simulink model "RobustFormationControl_IntegerModel_under_Dis"  (R2023a)
settings: Solver=ode3  StartTime=0.0  StopTime=30  FixedStep=0.0001  RelTol=1e-3
InitFcn:
  | % % Parameters for the fractional order NTFSMC:
  | % Sliding Surface " Sx, Sy, and Sz ":
  | %------------------------
  | % 10
  | % 10
  | cx = 2*[4 4 4];
  | cxx = 1*[0.01 0.01 0.01];
  | 
  | cx1 = cx(1);
  | cy1 = cx(2);
  | cz1 = cx(3);
  | 
  | cx2 = cxx(1);
  | cy2 = cxx(2);
  | cz2 = cxx(3);
  | 
  | alpha1 = [0.6 0.6 0.6];
  | alpha2 = [0.1 0.1 0.1];
  | 
  | gammaX = [3 3 3];
  | gx  = gammaX(1);
  | gy = gammaX(2);
  | gz = gammaX(3);
  | 
  | p = 10;
  | q = 10;
  | 
  | % Sliding Surface " S_Phi , S_Theta, and  S_Psi":
  | %------------------------
  | cP = 2*[4 4 4];
  | cPP = 1*[0.01 0.01 0.01 0.01];
  | 
  | cPhi1 = cP(1);
  | cTheta1 = cP(2);
  | cPsi1 = cP(3);
  | 
  | cPhi2 = cPP(1);
  | cTheta2 = cPP(2);
  | cPsi2 = cPP(3);
  | gammaP = [3 3 3];
  | 
  | %=========================
  | %=========================
  | SigmaX = 1*[0.01 0.01 0.01];
  | SigmaXX =1*[1 1 1];
  | 
  | Sigma1X = SigmaX(1);
  | Sigma1Y = SigmaX(2);
  | Sigma1Z = SigmaX(3);
  | %-----
  | Sigma2X = SigmaXX(1);
  | Sigma2Y = SigmaXX(2);
  | Sigma2Z = SigmaXX(3);
  | 
  | 
  | SigmaP = 1*[0.01 0.01 0.01];
  | SigmaPP =1*[1 1 1];
  | 
  | Sigma1Phi   = SigmaP(1);
  | Sigma1Theta = SigmaP(2);
  | ... (+80 lines)
values from neighbouring files (symbols this model uses):
  a1 = (Iyy - Izz)/Ixx    (= -0.812397034596)    [init_quadrotor_params.m]
  a2 = (Izz - Ixx)/Iyy    (= 0.812397034596)    [init_quadrotor_params.m]
  a3 = (Ixx - Iyy)/Izz    (= 0)    [init_quadrotor_params.m]
  a4 = - Ktx/m    (= -0.00114547325103)    [init_quadrotor_params.m]
  a5 = - Kty/m    (= -0.00114547325103)    [init_quadrotor_params.m]
  a6 = - Ktz/m    (= -0.00130740740741)    [init_quadrotor_params.m]
  b = 2.980e-5    (= 2.98e-05)    [init_quadrotor_params.m]
  b1 = - Jr/Ixx    (= -0.00584534596376)    [init_quadrotor_params.m]
  b2 = Jr/Iyy    (= 0.00584534596376)    [init_quadrotor_params.m]
  b3 = - Kfz/Izz    (= -0.0721963413248)    [init_quadrotor_params.m]
  b4 = 1/m    (= 2.05761316872)    [init_quadrotor_params.m]
  b5 = 1/m    (= 2.05761316872)    [init_quadrotor_params.m]
  b6 = 1/m    (= 2.05761316872)    [init_quadrotor_params.m]
  c1 = - Kfx/Ixx    (= -0.114641680395)    [init_quadrotor_params.m]
  c2 = - Kfy/Iyy    (= -0.114641680395)    [init_quadrotor_params.m]
  c3 = 1/Izz    (= 113.62345188)    [init_quadrotor_params.m]
  d = 1.12e-06    [init_quadrotor_params.m]
  d1 = L/Ixx    (= 46.334431631)    [init_quadrotor_params.m]
  d2 = L/Iyy    (= 46.334431631)    [init_quadrotor_params.m]
  g = 9.81    [init_quadrotor_params.m]
  Ixx = 4.856e-3    (= 0.004856)    [init_quadrotor_params.m]
  Iyy = 4.856e-3    (= 0.004856)    [init_quadrotor_params.m]
  Izz = 8.801e-3    (= 0.008801)    [init_quadrotor_params.m]
  Jr = 2.8385e-5    (= 2.8385e-05)    [init_quadrotor_params.m]
  Kfx = 5.567e-4    (= 0.0005567)    [init_quadrotor_params.m]
  Kfy = 5.567e-4    (= 0.0005567)    [init_quadrotor_params.m]
  Kfz = 6.354e-4    (= 0.0006354)    [init_quadrotor_params.m]
  Ktx = 5.5670e-4    (= 0.0005567)    [init_quadrotor_params.m]
  Kty = 5.5670e-4    (= 0.0005567)    [init_quadrotor_params.m]
  Ktz = 6.3540e-4    (= 0.0006354)    [init_quadrotor_params.m]
  L = 0.225    [init_quadrotor_params.m]
  m = 0.486    [init_quadrotor_params.m]
libraries: fod x120, eeStairGenerator x5
(part 9 of 9)

== system RobustFormationControl_IntegerModel_under_Dis/Integer Leader and four followers/Leader System/Integer Model/Control Module1/Subsystem/Subsystem1 ==
  Ux : Inport
  Uy : Inport  Port=2
  Psi_d : Inport  Port=3
  Phi_d : Inport  Port=4
  Constant : Constant
  Divide : Product  Inputs=*/
  Product : Product
  Product1 : Product
  Product2 : Product
  Subtract : Sum
  Trigonometric Function : Trigonometry  Operator=cos
  Trigonometric Function1 : Trigonometry
  Trigonometric Function2 : Trigonometry  Operator=asin
  Trigonometric Function3 : Trigonometry  Operator=cos
  Theta_d : Outport  VectorParamsAs1DForOutWhenUnconnected=off
  wires:
  Product1/1 -> Subtract/2
  Uy/1 -> Product1/2
  Ux/1 -> Product/1
  Trigonometric Function1/1 -> Product1/1
  Psi_d/1 -> Trigonometric Function1/1, Trigonometric Function/1
  Product/1 -> Subtract/1
  Trigonometric Function/1 -> Product/2
  Trigonometric Function2/1 -> Theta_d/1
  Constant/1 -> Divide/1
  Product2/1 -> Trigonometric Function2/1
  Subtract/1 -> Product2/1
  Divide/1 -> Product2/2
  Trigonometric Function3/1 -> Divide/2
  Phi_d/1 -> Trigonometric Function3/1

== system RobustFormationControl_IntegerModel_under_Dis/Integer Leader and four followers/Leader System/Integer Model/Control Module1/Subsystem1/Subsystem ==
  x1 : Inport
  xd1 : Inport  Port=2
  x2 : Inport  Port=3
  xd2 : Inport  Port=4
  Constant : Constant  Value=p/q
  Constant1 : Constant  Value=gammaP(1)
  Divide : Product  Inputs=**  RndMeth=Zero  SaturateOnIntegerOverflow=on
  Fractional integrator : fod/Fractional integrator  gam=0.01  ww=[0.001; 1000]  n=5  nFod=off
      settings: SourceProductName=FOMCON Toolbox
  Fractional integrator1 : fod/Fractional integrator  gam=0.01  ww=[0.001; 1000]  n=5  nFod=off
      settings: SourceProductName=FOMCON Toolbox
  Gain : Gain  Gain=cPhi1
  Gain1 : Gain  Gain=cPhi2
  Power : Math  Operator=pow
  Power1 : Math  Operator=pow
  Sign : Signum
  Sum1 : Sum  Inputs=+-
  Sum2 : Sum  Inputs=+++
  Sum3 : Sum  Inputs=+-
  S2 : Outport  VectorParamsAs1DForOutWhenUnconnected=off
  wires:
  xd2/1 -> Sum1/2
  Sum2/1 -> S2/1
  xd1/1 -> Sum3/2
  x1/1 -> Sum3/1
  x2/1 -> Sum1/1
  Sum3/1 -> Power1/1, Sign/1, Power/1
  Constant/1 -> Power/2
  Power/1 -> Gain/1
  Gain/1 -> Fractional integrator/1
  Constant1/1 -> Power1/2
  Sign/1 -> Divide/1
  Power1/1 -> Divide/2
  Divide/1 -> Gain1/1
  Gain1/1 -> Fractional integrator1/1
  Sum1/1 -> Sum2/1
  Fractional integrator/1 -> Sum2/2
  Fractional integrator1/1 -> Sum2/3

== system RobustFormationControl_IntegerModel_under_Dis/Integer Leader and four followers/Leader System/Integer Model/Control Module1/Subsystem1/Subsystem1 ==
  x5 : Inport
  xd5 : Inport  Port=2
  x6 : Inport  Port=3
  xd6 : Inport  Port=4
  Constant : Constant  Value=p/q
  Constant1 : Constant  Value=gammaP(3)
  Divide : Product  Inputs=**  RndMeth=Zero  SaturateOnIntegerOverflow=on
  Fractional integrator : fod/Fractional integrator  gam=0.1  ww=[0.001; 1000]  n=5  nFod=off
      settings: SourceProductName=FOMCON Toolbox
  Fractional integrator1 : fod/Fractional integrator  gam=0.1  ww=[0.001; 1000]  n=5  nFod=off
      settings: SourceProductName=FOMCON Toolbox
  Gain : Gain  Gain=cPsi1
  Gain1 : Gain  Gain=cPsi2
  Power : Math  Operator=pow
  Power1 : Math  Operator=pow
  Sign : Signum
  Sum1 : Sum  Inputs=+-
  Sum2 : Sum  Inputs=+++
  Sum3 : Sum  Inputs=+-
  S6 : Outport  VectorParamsAs1DForOutWhenUnconnected=off
  wires:
  xd6/1 -> Sum1/2
  Sum2/1 -> S6/1
  xd5/1 -> Sum3/2
  x5/1 -> Sum3/1
  x6/1 -> Sum1/1
  Sum3/1 -> Power1/1, Sign/1, Power/1
  Constant/1 -> Power/2
  Power/1 -> Gain/1
  Gain/1 -> Fractional integrator/1
  Constant1/1 -> Power1/2
  Sign/1 -> Divide/1
  Power1/1 -> Divide/2
  Divide/1 -> Gain1/1
  Gain1/1 -> Fractional integrator1/1
  Sum1/1 -> Sum2/1
  Fractional integrator/1 -> Sum2/2
  Fractional integrator1/1 -> Sum2/3

== system RobustFormationControl_IntegerModel_under_Dis/Integer Leader and four followers/Leader System/Integer Model/Control Module1/Subsystem1/Subsystem2 ==
  x7 : Inport
  xd7 : Inport  Port=2
  x8 : Inport  Port=3
  xd8 : Inport  Port=4
  Constant : Constant  Value=p/q
  Constant1 : Constant  Value=gx
  Divide : Product  Inputs=**  RndMeth=Zero  SaturateOnIntegerOverflow=on
  Fractional integrator : fod/Fractional integrator  gam=0.01  ww=[0.001; 1000]  n=5  nFod=off
      settings: SourceProductName=FOMCON Toolbox
  Fractional integrator1 : fod/Fractional integrator  gam=0.01  ww=[0.001; 1000]  n=5  nFod=off
      settings: SourceProductName=FOMCON Toolbox
  Gain : Gain  Gain=cx1
  Gain1 : Gain  Gain=cx2
  Power : Math  Operator=pow
  Power1 : Math  Operator=pow
  Sign : Signum
  Sum1 : Sum  Inputs=+-
  Sum2 : Sum  Inputs=+++
  Sum3 : Sum  Inputs=+-
  S8 : Outport  VectorParamsAs1DForOutWhenUnconnected=off
  wires:
  xd8/1 -> Sum1/2
  Sum2/1 -> S8/1
  xd7/1 -> Sum3/2
  x7/1 -> Sum3/1
  x8/1 -> Sum1/1
  Sum3/1 -> Power1/1, Sign/1, Power/1
  Constant/1 -> Power/2
  Power/1 -> Gain/1
  Gain/1 -> Fractional integrator/1
  Constant1/1 -> Power1/2
  Sign/1 -> Divide/1
  Power1/1 -> Divide/2
  Divide/1 -> Gain1/1
  Gain1/1 -> Fractional integrator1/1
  Sum1/1 -> Sum2/1
  Fractional integrator/1 -> Sum2/2
  Fractional integrator1/1 -> Sum2/3

== system RobustFormationControl_IntegerModel_under_Dis/Integer Leader and four followers/Leader System/Integer Model/Control Module1/Subsystem1/Subsystem3 ==
  x9 : Inport
  xd9 : Inport  Port=2
  x10 : Inport  Port=3
  xd10 : Inport  Port=4
  Constant : Constant  Value=p/q
  Constant1 : Constant  Value=gy
  Divide : Product  Inputs=**  RndMeth=Zero  SaturateOnIntegerOverflow=on
  Fractional integrator : fod/Fractional integrator  gam=0.1  ww=[0.001; 1000]  n=5  nFod=off
      settings: SourceProductName=FOMCON Toolbox
  Fractional integrator1 : fod/Fractional integrator  gam=0.1  ww=[0.001; 1000]  n=5  nFod=off
      settings: SourceProductName=FOMCON Toolbox
  Gain : Gain  Gain=cy1
  Gain1 : Gain  Gain=cy2
  Power : Math  Operator=pow
  Power1 : Math  Operator=pow
  Sign : Signum
  Sum1 : Sum  Inputs=+-
  Sum2 : Sum  Inputs=+++
  Sum3 : Sum  Inputs=+-
  S10 : Outport  VectorParamsAs1DForOutWhenUnconnected=off
  wires:
  xd10/1 -> Sum1/2
  Sum2/1 -> S10/1
  xd9/1 -> Sum3/2
  x9/1 -> Sum3/1
  x10/1 -> Sum1/1
  Sum3/1 -> Power1/1, Sign/1, Power/1
  Constant/1 -> Power/2
  Power/1 -> Gain/1
  Gain/1 -> Fractional integrator/1
  Constant1/1 -> Power1/2
  Sign/1 -> Divide/1
  Power1/1 -> Divide/2
  Divide/1 -> Gain1/1
  Gain1/1 -> Fractional integrator1/1
  Sum1/1 -> Sum2/1
  Fractional integrator/1 -> Sum2/2
  Fractional integrator1/1 -> Sum2/3

== system RobustFormationControl_IntegerModel_under_Dis/Integer Leader and four followers/Leader System/Integer Model/Control Module1/Subsystem1/Subsystem4 ==
  x11 : Inport
  xd11 : Inport  Port=2
  x12 : Inport  Port=3
  xd12 : Inport  Port=4
  Constant : Constant  Value=p/q
  Constant1 : Constant  Value=gz
  Divide : Product  Inputs=**  RndMeth=Zero  SaturateOnIntegerOverflow=on
  Fractional integrator : fod/Fractional integrator  gam=0.1  ww=[0.001; 1000]  n=5  nFod=off
      settings: SourceProductName=FOMCON Toolbox
  Fractional integrator1 : fod/Fractional integrator  gam=0.1  ww=[0.001; 1000]  n=5  nFod=off
      settings: SourceProductName=FOMCON Toolbox
  Gain : Gain  Gain=cz1
  Gain1 : Gain  Gain=cz2
  Power : Math  Operator=pow
  Power1 : Math  Operator=pow
  Sign : Signum
  Sum1 : Sum  Inputs=+-
  Sum2 : Sum  Inputs=+++
  Sum3 : Sum  Inputs=+-
  S12 : Outport  VectorParamsAs1DForOutWhenUnconnected=off
  wires:
  xd12/1 -> Sum1/2
  Sum2/1 -> S12/1
  xd11/1 -> Sum3/2
  x11/1 -> Sum3/1
  x12/1 -> Sum1/1
  Sum3/1 -> Power1/1, Sign/1, Power/1
  Constant/1 -> Power/2
  Power/1 -> Gain/1
  Gain/1 -> Fractional integrator/1
  Constant1/1 -> Power1/2
  Sign/1 -> Divide/1
  Power1/1 -> Divide/2
  Divide/1 -> Gain1/1
  Gain1/1 -> Fractional integrator1/1
  Sum1/1 -> Sum2/1
  Fractional integrator/1 -> Sum2/2
  Fractional integrator1/1 -> Sum2/3

== system RobustFormationControl_IntegerModel_under_Dis/Integer Leader and four followers/Leader System/Integer Model/Control Module1/Subsystem1/Subsystem6 ==
  x3 : Inport
  xd3 : Inport  Port=2
  x4 : Inport  Port=3
  xd4 : Inport  Port=4
  Constant : Constant  Value=p/q
  Constant1 : Constant  Value=gammaP(2)
  Divide : Product  Inputs=**  RndMeth=Zero  SaturateOnIntegerOverflow=on
  Fractional integrator : fod/Fractional integrator  gam=0.1  ww=[0.001; 1000]  n=5  nFod=off
      settings: SourceProductName=FOMCON Toolbox
  Fractional integrator1 : fod/Fractional integrator  gam=0.1  ww=[0.001; 1000]  n=5  nFod=off
      settings: SourceProductName=FOMCON Toolbox
  Gain : Gain  Gain=cTheta1
  Gain1 : Gain  Gain=cTheta2
  Power : Math  Operator=pow
  Power1 : Math  Operator=pow
  Sign : Signum
  Sum1 : Sum  Inputs=+-
  Sum2 : Sum  Inputs=+++
  Sum3 : Sum  Inputs=+-
  S4 : Outport  VectorParamsAs1DForOutWhenUnconnected=off
  wires:
  xd4/1 -> Sum1/2
  Sum2/1 -> S4/1
  xd3/1 -> Sum3/2
  x3/1 -> Sum3/1
  x4/1 -> Sum1/1
  Sum3/1 -> Power1/1, Sign/1, Power/1
  Constant/1 -> Power/2
  Power/1 -> Gain/1
  Gain/1 -> Fractional integrator/1
  Constant1/1 -> Power1/2
  Sign/1 -> Divide/1
  Power1/1 -> Divide/2
  Divide/1 -> Gain1/1
  Gain1/1 -> Fractional integrator1/1
  Sum1/1 -> Sum2/1
  Fractional integrator/1 -> Sum2/2
  Fractional integrator1/1 -> Sum2/3

== system RobustFormationControl_IntegerModel_under_Dis/Integer Leader and four followers/Leader System/Integer Model/Control Module1/Subsystem2/Subsystem ==
  x7 : Inport
  xd7 : Inport  Port=2
  x8 : Inport  Port=3
  xd8 : Inport  Port=4
  S8 : Inport  Port=5
  Constant : Constant  Value=q/p
  Constant1 : Constant  Value=gx-1
  Divide : Product  Inputs=**  RndMeth=Zero  SaturateOnIntegerOverflow=on
  Fractional derivative : fod/Fractional derivative  gam=alpha1(1)  ww=[0.001; 1000]  n=5  nFod=off
      settings: SourceProductName=FOMCON Toolbox
  Fractional integrator1 : fod/Fractional integrator  gam=alpha2(1)  ww=[0.001; 1000]  n=5  nFod=off
      settings: SourceProductName=FOMCON Toolbox
  Gain : Gain  Gain=cx1
  Gain1 : Gain  Gain=cx2
  Gain2 : Gain  Gain=gx
  Gain3 : Gain  Gain=Sigma1X
  Gain4 : Gain  Gain=Sigma2X
  Power : Math  Operator=pow
  Power1 : Math  Operator=pow
  Sign : Signum
  Sum : Sum
  Sum1 : Sum  Inputs=+-
  Sum2 : Sum  Inputs=---
  Sum3 : Sum  Inputs=+-
  D2 : Outport  VectorParamsAs1DForOutWhenUnconnected=off
  wires:
  xd8/1 -> Sum1/2
  xd7/1 -> Sum3/2
  x7/1 -> Sum3/1
  x8/1 -> Sum1/1
  Sum3/1 -> Power1/1, Power/1
  Constant/1 -> Power/2
  Power/1 -> Gain/1
  Gain/1 -> Fractional derivative/1
  Constant1/1 -> Power1/2
  Power1/1 -> Divide/2
  Divide/1 -> Gain1/1
  Gain1/1 -> Gain2/1
  Sum1/1 -> Divide/1
  Gain2/1 -> Fractional integrator1/1
  S8/1 -> Gain4/1, Sign/1
  Sign/1 -> Gain3/1
  Gain3/1 -> Sum/1
  Gain4/1 -> Sum/2
  Sum/1 -> Sum2/3
  Fractional derivative/1 -> Sum2/1
  Fractional integrator1/1 -> Sum2/2
  Sum2/1 -> D2/1

== system RobustFormationControl_IntegerModel_under_Dis/Integer Leader and four followers/Leader System/Integer Model/Control Module1/Subsystem2/Subsystem1 ==
  x8 : Inport
  x8d : Inport  Port=2
  Divide2 : Product  Inputs=**  RndMeth=Zero  SaturateOnIntegerOverflow=on
  Gain1 : Gain  Commented=on  Gain=a4
  Sum : Sum  Inputs=-+
  D1 : Outport
  wires:
  Sum/1 -> D1/1
  x8d/1 -> Sum/2
  [a4D] -> Divide2/1
  Divide2/1 -> Sum/1
  x8/1 -> Divide2/2

== system RobustFormationControl_IntegerModel_under_Dis/Integer Leader and four followers/Leader System/Integer Model/Control Module1/Subsystem2/Subsystem2 ==
  x7 : Inport
  xd7 : Inport  Port=2
  x8 : Inport  Port=3
  xd8 : Inport  Port=4
  S8 : Inport  Port=5
  Abs : Abs  SaturateOnIntegerOverflow=off
  Divide{,1..4} (5 alike) : Product  Inputs=**  RndMeth=Zero  SaturateOnIntegerOverflow=on
  Gain : Gain  Gain=q0
  Gain1 : Gain  Gain=q1
  Gain2 : Gain  Gain=q2
  Integrator : Integrator
  Integrator1 : Integrator
  Integrator2 : Integrator
  Mux : Mux  Inputs=3
  Scope : Scope
  Scope1 : Scope
  Scope2 : Scope
  Sign : Signum
  Sum1 : Sum  Inputs=+-
  Sum2 : Sum  Inputs=----
  Sum3 : Sum  Inputs=+-
  To Workspace : ToWorkspace  VariableName=Bx  SampleTime=-1
  w : Constant  Value=w
  D3 : Outport  VectorParamsAs1DForOutWhenUnconnected=off
  wires:
  xd8/1 -> Sum1/2
  xd7/1 -> Sum3/2
  x7/1 -> Sum3/1
  x8/1 -> Sum1/1
  S8/1 -> [S8], Abs/1
  Sum1/1 -> [e2]
  Sum3/1 -> [e1]
  Gain/1 -> Integrator/1
  Integrator/1 -> Scope/1, Mux/1, Sum2/1  "B0"
  [e1] -> Divide/2
  Gain1/1 -> Integrator1/1
  Divide/1 -> Gain1/1
  Divide1/1 -> Gain2/1
  Gain2/1 -> Integrator2/1
  [e2] -> Divide1/2
  Abs/1 -> Divide1/1, Divide/1, Gain/1
  Integrator1/1 -> Scope1/1, Divide3/2  "B1"
  w/1 -> Sum2/4
  Sign/1 -> Divide2/2
  [S8] -> Sign/1
  Divide2/1 -> D3/1
  [e1] -> Divide3/1
  [e2] -> Divide4/1
  Integrator2/1 -> Divide4/2, Scope2/1  "B2"
  Divide3/1 -> Mux/2, Sum2/2
  Divide4/1 -> Mux/3, Sum2/3
  Sum2/1 -> Divide2/1
  Mux/1 -> To Workspace/1

== system RobustFormationControl_IntegerModel_under_Dis/Integer Leader and four followers/Leader System/Integer Model/Control Module1/Subsystem3/Subsystem ==
  x9 : Inport
  xd9 : Inport  Port=2
  x10 : Inport  Port=3
  xd10 : Inport  Port=4
  S10 : Inport  Port=5
  Constant : Constant  Value=p/q
  Constant1 : Constant  Value=gy-1
  Divide : Product  Inputs=**  RndMeth=Zero  SaturateOnIntegerOverflow=on
  Fractional derivative : fod/Fractional derivative  gam=alpha1(2)  ww=[0.001; 1000]  n=5  nFod=off
      settings: SourceProductName=FOMCON Toolbox
  Fractional integrator1 : fod/Fractional integrator  gam=alpha2(2)  ww=[0.001; 1000]  n=5  nFod=off
      settings: SourceProductName=FOMCON Toolbox
  Gain : Gain  Gain=cy1
  Gain1 : Gain  Gain=gy
  Gain2 : Gain  Gain=cy2
  Gain3 : Gain  Gain=Sigma1Y
  Gain4 : Gain  Gain=Sigma2Y
  Power : Math  Operator=pow
  Power1 : Math  Operator=pow
  Sign : Signum
  Sum : Sum
  Sum1 : Sum  Inputs=+-
  Sum2 : Sum  Inputs=---
  Sum3 : Sum  Inputs=+-
  D2 : Outport  VectorParamsAs1DForOutWhenUnconnected=off
  wires:
  xd10/1 -> Sum1/2
  xd9/1 -> Sum3/2
  x9/1 -> Sum3/1
  x10/1 -> Sum1/1
  Sum3/1 -> Power1/1, Power/1
  Constant/1 -> Power/2
  Power/1 -> Gain/1
  Gain/1 -> Fractional derivative/1
  Constant1/1 -> Power1/2
  Power1/1 -> Divide/2
  Divide/1 -> Gain1/1
  Gain1/1 -> Gain2/1
  Sum1/1 -> Divide/1
  Gain2/1 -> Fractional integrator1/1
  S10/1 -> Gain4/1, Sign/1
  Sign/1 -> Gain3/1
  Gain3/1 -> Sum/1
  Gain4/1 -> Sum/2
  Sum/1 -> Sum2/3
  Fractional derivative/1 -> Sum2/1
  Fractional integrator1/1 -> Sum2/2
  Sum2/1 -> D2/1

== system RobustFormationControl_IntegerModel_under_Dis/Integer Leader and four followers/Leader System/Integer Model/Control Module1/Subsystem3/Subsystem1 ==
  x10 : Inport
  x10d : Inport  Port=2
  Divide2 : Product  Inputs=**  RndMeth=Zero  SaturateOnIntegerOverflow=on
  Gain1 : Gain  Commented=on  Gain=a5
  Sum : Sum  Inputs=-+
  D1 : Outport
  wires:
  Sum/1 -> D1/1
  x10d/1 -> Sum/2
  [a5D] -> Divide2/1
  Divide2/1 -> Sum/1
  x10/1 -> Divide2/2

== system RobustFormationControl_IntegerModel_under_Dis/Integer Leader and four followers/Leader System/Integer Model/Control Module1/Subsystem3/Subsystem2 ==
  x9 : Inport
  xd9 : Inport  Port=2
  x10 : Inport  Port=3
  xd10 : Inport  Port=4
  S10 : Inport  Port=5
  Abs : Abs  SaturateOnIntegerOverflow=off
  Divide{,1..4} (5 alike) : Product  Inputs=**  RndMeth=Zero  SaturateOnIntegerOverflow=on
  Gain : Gain  Gain=q0
  Gain1 : Gain  Gain=q1
  Gain2 : Gain  Gain=q2
  Integrator : Integrator
  Integrator1 : Integrator
  Integrator2 : Integrator
  Mux : Mux  Inputs=3
  Sign : Signum
  Sum1 : Sum  Inputs=+-
  Sum2 : Sum  Inputs=----
  Sum3 : Sum  Inputs=+-
  To Workspace : ToWorkspace  VariableName=By  SampleTime=-1
  w : Constant  Value=w
  D3 : Outport  VectorParamsAs1DForOutWhenUnconnected=off
  wires:
  xd10/1 -> Sum1/2
  xd9/1 -> Sum3/2
  x9/1 -> Sum3/1
  x10/1 -> Sum1/1
  S10/1 -> [S10], Abs/1
  Sum1/1 -> [e2]
  Sum3/1 -> [e1]
  Gain/1 -> Integrator/1
  [e1] -> Divide/2
  Gain1/1 -> Integrator1/1
  Divide/1 -> Gain1/1
  Divide1/1 -> Gain2/1
  Gain2/1 -> Integrator2/1
  [e2] -> Divide1/2
  Abs/1 -> Divide1/1, Divide/1, Gain/1
  Integrator1/1 -> Divide3/2  "B1"
  w/1 -> Sum2/4
  Sign/1 -> Divide2/2
  [S10] -> Sign/1
  Divide2/1 -> D3/1
  [e1] -> Divide3/1
  [e2] -> Divide4/1
  Integrator2/1 -> Divide4/2  "B2"
  Sum2/1 -> Divide2/1
  Mux/1 -> To Workspace/1
  Divide4/1 -> Mux/3, Sum2/3
  Integrator/1 -> Mux/1, Sum2/1  "B0"
  Divide3/1 -> Mux/2, Sum2/2

== system RobustFormationControl_IntegerModel_under_Dis/Integer Leader and four followers/Leader System/Integer Model/Control Module1/Subsystem4/Subsystem ==
  x1 : Inport
  xd1 : Inport  Port=2
  x2 : Inport  Port=3
  xd2 : Inport  Port=4
  S2 : Inport  Port=5
  Constant : Constant  Value=p/q
  Constant1 : Constant  Value=gammaP(1)-1
  Divide : Product  Inputs=**  RndMeth=Zero  SaturateOnIntegerOverflow=on
  Fractional derivative : fod/Fractional derivative  gam=alpha1(1)  ww=[0.001; 1000]  n=5  nFod=off
      settings: SourceProductName=FOMCON Toolbox
  Fractional integrator1 : fod/Fractional integrator  gam=alpha2(2)  ww=[0.001; 1000]  n=5  nFod=off
      settings: SourceProductName=FOMCON Toolbox
  Gain : Gain  Gain=cPhi1
  Gain1 : Gain  Gain=cPhi2
  Gain2 : Gain  Gain=gammaP(1)
  Gain3 : Gain  Gain=Sigma1Phi
  Gain4 : Gain  Gain=Sigma1Phi
  Power : Math  Operator=pow
  Power1 : Math  Operator=pow
  Sign : Signum
  Sum : Sum
  Sum1 : Sum  Inputs=+-
  Sum2 : Sum  Inputs=---
  Sum3 : Sum  Inputs=+-
  D2 : Outport  VectorParamsAs1DForOutWhenUnconnected=off
  wires:
  xd2/1 -> Sum1/2
  xd1/1 -> Sum3/2
  x1/1 -> Sum3/1
  x2/1 -> Sum1/1
  Sum3/1 -> Power1/1, Power/1
  Constant/1 -> Power/2
  Power/1 -> Gain/1
  Gain/1 -> Fractional derivative/1
  Constant1/1 -> Power1/2
  Power1/1 -> Divide/2
  Divide/1 -> Gain1/1
  Gain1/1 -> Gain2/1
  Sum1/1 -> Divide/1
  Gain2/1 -> Fractional integrator1/1
  S2/1 -> Gain4/1, Sign/1
  Sign/1 -> Gain3/1
  Gain3/1 -> Sum/1
  Gain4/1 -> Sum/2
  Sum/1 -> Sum2/3
  Fractional derivative/1 -> Sum2/1
  Fractional integrator1/1 -> Sum2/2
  Sum2/1 -> D2/1

== system RobustFormationControl_IntegerModel_under_Dis/Integer Leader and four followers/Leader System/Integer Model/Control Module1/Subsystem4/Subsystem1 ==
  x4 : Inport
  x6 : Inport  Port=2
  x2 : Inport  Port=3
  Omega : Inport  Port=4
  xd2 : Inport  Port=5
  Gain : Gain  Commented=on  Gain=a1
  Gain6 : Gain  Commented=on  Gain=c1
  Gain7 : Gain  Commented=on  Gain=b1
  Math Function : Math  Operator=square  SignedPower=on
  Product{,1..4} (5 alike) : Product
  Sum3 : Sum  Inputs=---+
  D1 : Outport
  wires:
  xd2/1 -> Sum3/4
  Product1/1 -> Product/2
  Sum3/1 -> D1/1
  Product2/1 -> Sum3/2  "c1 x2^2"
  Product4/1 -> Sum3/3
  Product3/1 -> Product4/2
  Omega/1 -> Product3/2
  Math Function/1 -> Product2/2  "x2^2"
  x4/1 -> Product3/1, Product1/1
  Product/1 -> Sum3/1  "a1 x4 x6"
  x6/1 -> Product1/2
  x2/1 -> Math Function/1
  [a1D] -> Product/1
  [c1D] -> Product2/1
  [b1D] -> Product4/1

== system RobustFormationControl_IntegerModel_under_Dis/Integer Leader and four followers/Leader System/Integer Model/Control Module1/Subsystem4/Subsystem2 ==
  x1 : Inport
  xd1 : Inport  Port=2
  x2 : Inport  Port=3
  xd2 : Inport  Port=4
  S2 : Inport  Port=5
  Abs : Abs  SaturateOnIntegerOverflow=off
  Divide{,1..4} (5 alike) : Product  Inputs=**  RndMeth=Zero  SaturateOnIntegerOverflow=on
  Gain : Gain  Gain=q0
  Gain1 : Gain  Gain=q1
  Gain2 : Gain  Gain=q2
  Integrator : Integrator
  Integrator1 : Integrator
  Integrator2 : Integrator
  Sign : Signum
  Sum1 : Sum  Inputs=+-
  Sum2 : Sum  Inputs=----
  Sum3 : Sum  Inputs=+-
  w : Constant  Value=w
  D3 : Outport  VectorParamsAs1DForOutWhenUnconnected=off
  wires:
  xd2/1 -> Sum1/2
  xd1/1 -> Sum3/2
  x1/1 -> Sum3/1
  x2/1 -> Sum1/1
  S2/1 -> [S2], Abs/1
  Sum1/1 -> [e2]
  Sum3/1 -> [e1]
  Gain/1 -> Integrator/1
  Integrator/1 -> Sum2/1  "B0"
  [e1] -> Divide/2
  Gain1/1 -> Integrator1/1
  Divide/1 -> Gain1/1
  Divide1/1 -> Gain2/1
  Gain2/1 -> Integrator2/1
  [e2] -> Divide1/2
  Abs/1 -> Divide1/1, Divide/1, Gain/1
  Integrator1/1 -> Divide3/2  "B1"
  w/1 -> Sum2/4
  Sign/1 -> Divide2/2
  [S2] -> Sign/1
  Divide2/1 -> D3/1
  [e1] -> Divide3/1
  [e2] -> Divide4/1
  Integrator2/1 -> Divide4/2  "B2"
  Divide3/1 -> Sum2/2
  Divide4/1 -> Sum2/3
  Sum2/1 -> Divide2/1

== system RobustFormationControl_IntegerModel_under_Dis/Integer Leader and four followers/Leader System/Integer Model/Control Module1/Subsystem5/Subsystem ==
  x5 : Inport
  xd5 : Inport  Port=2
  x6 : Inport  Port=3
  xd6 : Inport  Port=4
  S4 : Inport  Port=5
  Constant : Constant  Value=p/q
  Constant1 : Constant  Value=gammaP(3)-1
  Divide : Product  Inputs=**  RndMeth=Zero  SaturateOnIntegerOverflow=on
  Fractional derivative : fod/Fractional derivative  gam=alpha1(3)  ww=[0.001; 1000]  n=5  nFod=off
      settings: SourceProductName=FOMCON Toolbox
  Fractional integrator1 : fod/Fractional integrator  gam=alpha2(2)  ww=[0.001; 1000]  n=5  nFod=off
      settings: SourceProductName=FOMCON Toolbox
  Gain : Gain  Gain=cPsi1
  Gain1 : Gain  Gain=cPsi2
  Gain2 : Gain  Gain=gammaP(3)
  Gain3 : Gain  Gain=Sigma1Psi
  Gain4 : Gain  Gain=Sigma2Psi
  Power : Math  Operator=pow
  Power1 : Math  Operator=pow
  Sign : Signum
  Sum : Sum
  Sum1 : Sum  Inputs=+-
  Sum2 : Sum  Inputs=---
  Sum3 : Sum  Inputs=+-
  D2 : Outport  VectorParamsAs1DForOutWhenUnconnected=off
  wires:
  xd6/1 -> Sum1/2
  xd5/1 -> Sum3/2
  x5/1 -> Sum3/1
  x6/1 -> Sum1/1
  Sum3/1 -> Power1/1, Power/1
  Constant/1 -> Power/2
  Power/1 -> Gain/1
  Gain/1 -> Fractional derivative/1
  Constant1/1 -> Power1/2
  Power1/1 -> Divide/2
  Divide/1 -> Gain1/1
  Gain1/1 -> Gain2/1
  Sum1/1 -> Divide/1
  Gain2/1 -> Fractional integrator1/1
  S4/1 -> Gain4/1, Sign/1
  Sign/1 -> Gain3/1
  Gain3/1 -> Sum/1
  Gain4/1 -> Sum/2
  Sum/1 -> Sum2/3
  Fractional derivative/1 -> Sum2/1
  Fractional integrator1/1 -> Sum2/2
  Sum2/1 -> D2/1

== system RobustFormationControl_IntegerModel_under_Dis/Integer Leader and four followers/Leader System/Integer Model/Control Module1/Subsystem5/Subsystem1 ==
  x4 : Inport
  x6 : Inport  Port=2
  x2 : Inport  Port=3
  xd6 : Inport  Port=4
  Gain : Gain  Commented=on  Gain=a3
  Gain6 : Gain  Commented=on  Gain=b3
  Math Function : Math  Operator=square  SignedPower=on
  Product : Product
  Product1 : Product
  Product2 : Product
  Sum1 : Sum  Inputs=--+
  D1 : Outport
  wires:
  x6/1 -> Math Function/1
  Product1/1 -> Product/2
  xd6/1 -> Sum1/3
  Product2/1 -> Sum1/2  "c1 x2^2"
  Math Function/1 -> Product2/2  "x2^2"
  x2/1 -> Product1/1
  Product/1 -> Sum1/1  "a1 x4 x6"
  x4/1 -> Product1/2
  Sum1/1 -> D1/1
  [a3D] -> Product/1
  [b3D] -> Product2/1

== system RobustFormationControl_IntegerModel_under_Dis/Integer Leader and four followers/Leader System/Integer Model/Control Module1/Subsystem5/Subsystem2 ==
  x5 : Inport
  xd5 : Inport  Port=2
  x6 : Inport  Port=3
  xd6 : Inport  Port=4
  S6 : Inport  Port=5
  Abs : Abs  SaturateOnIntegerOverflow=off
  Divide{,1..4} (5 alike) : Product  Inputs=**  RndMeth=Zero  SaturateOnIntegerOverflow=on
  Gain : Gain  Gain=q0
  Gain1 : Gain  Gain=q1
  Gain2 : Gain  Gain=q2
  Integrator : Integrator
  Integrator1 : Integrator
  Integrator2 : Integrator
  Sign : Signum
  Sum1 : Sum  Inputs=+-
  Sum2 : Sum  Inputs=----
  Sum3 : Sum  Inputs=+-
  w : Constant  Value=w
  D3 : Outport  VectorParamsAs1DForOutWhenUnconnected=off
  wires:
  xd6/1 -> Sum1/2
  xd5/1 -> Sum3/2
  x5/1 -> Sum3/1
  x6/1 -> Sum1/1
  S6/1 -> [S6], Abs/1
  Sum1/1 -> [e2]
  Sum3/1 -> [e1]
  Gain/1 -> Integrator/1
  Integrator/1 -> Sum2/1  "B0"
  [e1] -> Divide/2
  Gain1/1 -> Integrator1/1
  Divide/1 -> Gain1/1
  Divide1/1 -> Gain2/1
  Gain2/1 -> Integrator2/1
  [e2] -> Divide1/2
  Abs/1 -> Divide1/1, Divide/1, Gain/1
  Integrator1/1 -> Divide3/2  "B1"
  w/1 -> Sum2/4
  Sign/1 -> Divide2/2
  [S6] -> Sign/1
  Divide2/1 -> D3/1
  [e1] -> Divide3/1
  [e2] -> Divide4/1
  Integrator2/1 -> Divide4/2  "B2"
  Divide3/1 -> Sum2/2
  Divide4/1 -> Sum2/3
  Sum2/1 -> Divide2/1

== system RobustFormationControl_IntegerModel_under_Dis/Integer Leader and four followers/Leader System/Integer Model/Control Module1/Subsystem6/Subsystem ==
  x11 : Inport
  xd11 : Inport  Port=2
  x12 : Inport  Port=3
  xd12 : Inport  Port=4
  S12 : Inport  Port=5
  Constant : Constant  Value=p/q
  Constant1 : Constant  Value=gz-1
  Divide : Product  Inputs=**  RndMeth=Zero  SaturateOnIntegerOverflow=on
  Fractional derivative : fod/Fractional derivative  gam=alpha1(3)  ww=[0.001; 1000]  n=5  nFod=off
      settings: SourceProductName=FOMCON Toolbox
  Fractional integrator1 : fod/Fractional integrator  gam=alpha2(3)  ww=[0.001; 1000]  n=5  nFod=off
      settings: SourceProductName=FOMCON Toolbox
  Gain : Gain  Gain=cz1
  Gain1 : Gain  Gain=cz2
  Gain2 : Gain  Gain=gz
  Gain3 : Gain  Gain=Sigma1Z
  Gain4 : Gain  Gain=Sigma2Z
  Power : Math  Operator=pow
  Power1 : Math  Operator=pow
  Sign : Signum
  Sum : Sum
  Sum1 : Sum  Inputs=+-
  Sum2 : Sum  Inputs=---
  Sum3 : Sum  Inputs=+-
  D2 : Outport  VectorParamsAs1DForOutWhenUnconnected=off
  wires:
  xd12/1 -> Sum1/2
  xd11/1 -> Sum3/2
  x11/1 -> Sum3/1
  x12/1 -> Sum1/1
  Sum3/1 -> Power1/1, Power/1
  Constant/1 -> Power/2
  Power/1 -> Gain/1
  Gain/1 -> Fractional derivative/1
  Constant1/1 -> Power1/2
  Power1/1 -> Divide/2
  Divide/1 -> Gain1/1
  Gain1/1 -> Gain2/1
  Sum1/1 -> Divide/1
  Gain2/1 -> Fractional integrator1/1
  S12/1 -> Gain4/1, Sign/1
  Sign/1 -> Gain3/1
  Gain3/1 -> Sum/1
  Gain4/1 -> Sum/2
  Sum/1 -> Sum2/3
  Fractional derivative/1 -> Sum2/1
  Fractional integrator1/1 -> Sum2/2
  Sum2/1 -> D2/1

== system RobustFormationControl_IntegerModel_under_Dis/Integer Leader and four followers/Leader System/Integer Model/Control Module1/Subsystem6/Subsystem1 ==
  x12 : Inport
  x12d : Inport  Port=2
  Constant2 : Constant  Value=g
  Divide2 : Product  Inputs=**  RndMeth=Zero  SaturateOnIntegerOverflow=on
  Gain1 : Gain  Commented=on  Gain=a6
  Sum : Sum  Inputs=-++
  D1 : Outport
  wires:
  Sum/1 -> D1/1
  x12/1 -> Divide2/2
  Divide2/1 -> Sum/1
  Constant2/1 -> Sum/2
  x12d/1 -> Sum/3
  [a6D] -> Divide2/1

== system RobustFormationControl_IntegerModel_under_Dis/Integer Leader and four followers/Leader System/Integer Model/Control Module1/Subsystem6/Subsystem2 ==
  x11 : Inport
  xd11 : Inport  Port=2
  x12 : Inport  Port=3
  xd12 : Inport  Port=4
  S12 : Inport  Port=5
  Abs : Abs  SaturateOnIntegerOverflow=off
  Divide{,1..4} (5 alike) : Product  Inputs=**  RndMeth=Zero  SaturateOnIntegerOverflow=on
  Gain : Gain  Gain=q0
  Gain1 : Gain  Gain=q1
  Gain2 : Gain  Gain=q2
  Integrator : Integrator
  Integrator1 : Integrator
  Integrator2 : Integrator
  Mux : Mux  Inputs=3
  Sign : Signum
  Sum1 : Sum  Inputs=+-
  Sum2 : Sum  Inputs=----
  Sum3 : Sum  Inputs=+-
  To Workspace : ToWorkspace  VariableName=Bz  SampleTime=-1
  w : Constant  Value=w
  D3 : Outport  VectorParamsAs1DForOutWhenUnconnected=off
  wires:
  xd12/1 -> Sum1/2
  xd11/1 -> Sum3/2
  x11/1 -> Sum3/1
  x12/1 -> Sum1/1
  S12/1 -> [S12], Abs/1
  Sum1/1 -> [e2]
  Sum3/1 -> [e1]
  Gain/1 -> Integrator/1
  [e1] -> Divide/2
  Gain1/1 -> Integrator1/1
  Divide/1 -> Gain1/1
  Divide1/1 -> Gain2/1
  Gain2/1 -> Integrator2/1
  [e2] -> Divide1/2
  Abs/1 -> Divide1/1, Divide/1, Gain/1
  Integrator1/1 -> Divide3/2  "B1"
  w/1 -> Sum2/4
  Sign/1 -> Divide2/2
  [S12] -> Sign/1
  Divide2/1 -> D3/1
  [e1] -> Divide3/1
  [e2] -> Divide4/1
  Integrator2/1 -> Divide4/2  "B2"
  Sum2/1 -> Divide2/1
  Mux/1 -> To Workspace/1
  Divide4/1 -> Mux/3, Sum2/3
  Integrator/1 -> Mux/1, Sum2/1  "B0"
  Divide3/1 -> Mux/2, Sum2/2

== system RobustFormationControl_IntegerModel_under_Dis/Integer Leader and four followers/Leader System/Integer Model/Control Module1/Subsystem8/Subsystem ==
  x3 : Inport
  xd3 : Inport  Port=2
  x4 : Inport  Port=3
  xd4 : Inport  Port=4
  S4 : Inport  Port=5
  Constant : Constant  Value=p/q
  Constant1 : Constant  Value=gammaP(2)-1
  Divide : Product  Inputs=**  RndMeth=Zero  SaturateOnIntegerOverflow=on
  Fractional derivative : fod/Fractional derivative  gam=alpha1(2)  ww=[0.001; 1000]  n=5  nFod=off
      settings: SourceProductName=FOMCON Toolbox
  Fractional integrator1 : fod/Fractional integrator  gam=alpha2(2)  ww=[0.001; 1000]  n=5  nFod=off
      settings: SourceProductName=FOMCON Toolbox
  Gain : Gain  Gain=cTheta1
  Gain1 : Gain  Gain=cTheta2
  Gain2 : Gain  Gain=gammaP(2)
  Gain3 : Gain  Gain=Sigma1Theta
  Gain4 : Gain  Gain=Sigma2Theta
  Power : Math  Operator=pow
  Power1 : Math  Operator=pow
  Sign : Signum
  Sum : Sum
  Sum1 : Sum  Inputs=+-
  Sum2 : Sum  Inputs=---
  Sum3 : Sum  Inputs=+-
  D2 : Outport  VectorParamsAs1DForOutWhenUnconnected=off
  wires:
  xd4/1 -> Sum1/2
  xd3/1 -> Sum3/2
  x3/1 -> Sum3/1
  x4/1 -> Sum1/1
  Sum3/1 -> Power1/1, Power/1
  Constant/1 -> Power/2
  Power/1 -> Gain/1
  Gain/1 -> Fractional derivative/1
  Constant1/1 -> Power1/2
  Power1/1 -> Divide/2
  Divide/1 -> Gain1/1
  Gain1/1 -> Gain2/1
  Sum1/1 -> Divide/1
  Gain2/1 -> Fractional integrator1/1
  S4/1 -> Gain4/1, Sign/1
  Sign/1 -> Gain3/1
  Gain3/1 -> Sum/1
  Gain4/1 -> Sum/2
  Sum/1 -> Sum2/3
  Fractional derivative/1 -> Sum2/1
  Fractional integrator1/1 -> Sum2/2
  Sum2/1 -> D2/1

== system RobustFormationControl_IntegerModel_under_Dis/Integer Leader and four followers/Leader System/Integer Model/Control Module1/Subsystem8/Subsystem1 ==
  x4 : Inport
  x6 : Inport  Port=2
  x2 : Inport  Port=3
  Omega : Inport  Port=4
  xd4 : Inport  Port=5
  Gain1 : Gain  Commented=on  Gain=a2
  Gain2 : Gain  Commented=on  Gain=c2
  Gain3 : Gain  Commented=on  Gain=b2
  Math Function1 : Math  Operator=square  SignedPower=on
  Product{,1..4} (5 alike) : Product
  Sum3 : Sum  Inputs=---+
  D1 : Outport
  wires:
  x6/1 -> Product2/2
  Product/1 -> Sum3/1  "a1 x4 x6"
  Sum3/1 -> D1/1
  Math Function1/1 -> Product1/2  "x2^2"
  x2/1 -> Product4/1, Product2/1
  x4/1 -> Math Function1/1
  xd4/1 -> Sum3/4
  Product4/1 -> Product3/2
  Omega/1 -> Product4/2
  Product2/1 -> Product/2
  Product3/1 -> Sum3/3
  Product1/1 -> Sum3/2  "c1 x2^2"
  [a2D] -> Product/1
  [c2D] -> Product1/1
  [b2D] -> Product3/1

== system RobustFormationControl_IntegerModel_under_Dis/Integer Leader and four followers/Leader System/Integer Model/Control Module1/Subsystem8/Subsystem2 ==
  x3 : Inport
  xd3 : Inport  Port=2
  x4 : Inport  Port=3
  xd4 : Inport  Port=4
  S4 : Inport  Port=5
  Abs : Abs  SaturateOnIntegerOverflow=off
  Divide{,1..4} (5 alike) : Product  Inputs=**  RndMeth=Zero  SaturateOnIntegerOverflow=on
  Gain : Gain  Gain=q0
  Gain1 : Gain  Gain=q1
  Gain2 : Gain  Gain=q2
  Integrator : Integrator
  Integrator1 : Integrator
  Integrator2 : Integrator
  Sign : Signum
  Sum1 : Sum  Inputs=+-
  Sum2 : Sum  Inputs=----
  Sum3 : Sum  Inputs=+-
  w : Constant  Value=w
  D3 : Outport  VectorParamsAs1DForOutWhenUnconnected=off
  wires:
  xd4/1 -> Sum1/2
  xd3/1 -> Sum3/2
  x3/1 -> Sum3/1
  x4/1 -> Sum1/1
  S4/1 -> [S4], Abs/1
  Sum1/1 -> [e2]
  Sum3/1 -> [e1]
  Gain/1 -> Integrator/1
  Integrator/1 -> Sum2/1  "B0"
  [e1] -> Divide/2
  Gain1/1 -> Integrator1/1
  Divide/1 -> Gain1/1
  Divide1/1 -> Gain2/1
  Gain2/1 -> Integrator2/1
  [e2] -> Divide1/2
  Abs/1 -> Divide1/1, Divide/1, Gain/1
  Integrator1/1 -> Divide3/2  "B1"
  w/1 -> Sum2/4
  Sign/1 -> Divide2/2
  [S4] -> Sign/1
  Divide2/1 -> D3/1
  [e1] -> Divide3/1
  [e2] -> Divide4/1
  Integrator2/1 -> Divide4/2  "B2"
  Divide3/1 -> Sum2/2
  Divide4/1 -> Sum2/3
  Sum2/1 -> Divide2/1

== system RobustFormationControl_IntegerModel_under_Dis/Integer Leader and four followers/Leader System/Integer Model/Quadrotor Dynamic System/Rotational System/Equation1 ==
  x4 : Inport
  x6 : Inport  Port=2
  U2 : Inport  Port=3
  Omega : Inport  Port=4
  Gain : Gain  Commented=on  Gain=a1
  Gain1 : Gain  Commented=on  Gain=c1
  Gain2 : Gain  Commented=on  Gain=b1
  Gain3 : Gain  Commented=on  Gain=d1
  Gain4 : Gain
  Gain5 : Gain  Gain=Dis
  Integrator : Integrator
  Integrator1 : Integrator
  Math Function : Math  Operator=square  SignedPower=on
  Product{,1..5} (6 alike) : Product
  Sum : Sum  Inputs=|++++
  Sum1 : Sum
  x1 = Phi : Outport  VectorParamsAs1DForOutWhenUnconnected=off
  x2 : Outport  Port=2  VectorParamsAs1DForOutWhenUnconnected=off
  wires:
  Math Function/1 -> Product4/2  "x2^2"
  x4/1 -> Product1/1, Product/1
  Integrator/1 -> Math Function/1, x2/1, Integrator1/1
  U2/1 -> Product5/2
  Product3/1 -> Sum/3
  Product5/1 -> Sum/4
  Product2/1 -> Sum/1  "a1 x4 x6"
  Product1/1 -> Product3/2
  Product4/1 -> Sum/2  "c1 x2^2"
  Integrator1/1 -> x1 = Phi/1
  Product/1 -> Product2/2
  x6/1 -> Product/2
  Omega/1 -> Product1/2
  Sum1/1 -> Integrator/1
  [Dphi1] -> Gain5/1
  Sum/1 -> Sum1/2
  Gain4/1 -> Sum1/1
  Gain5/1 -> Gain4/1
  [a1D] -> Product2/1
  [b1D] -> Product3/1
  [c1D] -> Product4/1
  [d1D] -> Product5/1

== system RobustFormationControl_IntegerModel_under_Dis/Integer Leader and four followers/Leader System/Integer Model/Quadrotor Dynamic System/Rotational System/Equation2 ==
  x2 : Inport
  x6 : Inport  Port=2
  U3 : Inport  Port=3
  Omega : Inport  Port=4
  Gain : Gain  Commented=on  Gain=a2
  Gain1 : Gain  Commented=on  Gain=c2
  Gain2 : Gain  Commented=on  Gain=b2
  Gain3 : Gain  Commented=on  Gain=d2
  Gain4 : Gain
  Gain5 : Gain  Gain=Dis
  Integrator : Integrator
  Integrator1 : Integrator
  Math Function : Math  Operator=square  SignedPower=on
  Product{,1..5} (6 alike) : Product
  Sum : Sum  Inputs=|++++
  Sum1 : Sum
  x3 =Theta : Outport  VectorParamsAs1DForOutWhenUnconnected=off
  x4 : Outport  Port=2  VectorParamsAs1DForOutWhenUnconnected=off
  wires:
  Math Function/1 -> Product4/2  "x4^2"
  x2/1 -> Product1/1, Product/1
  Integrator/1 -> Math Function/1, x4/1, Integrator1/1
  U3/1 -> Product5/2
  Product3/1 -> Sum/3
  Product5/1 -> Sum/4
  Product2/1 -> Sum/1  "a2 x2 x6"
  Product1/1 -> Product3/2
  Product4/1 -> Sum/2  "c2 x2^2"
  Integrator1/1 -> x3 =Theta/1
  Product/1 -> Product2/2
  x6/1 -> Product/2
  Omega/1 -> Product1/2
  Sum1/1 -> Integrator/1
  [Dphi2] -> Gain5/1
  Sum/1 -> Sum1/2
  Gain4/1 -> Sum1/1
  Gain5/1 -> Gain4/1
  [a2D] -> Product2/1
  [b2D] -> Product3/1
  [c2D] -> Product4/1
  [d2D] -> Product5/1

== system RobustFormationControl_IntegerModel_under_Dis/Integer Leader and four followers/Leader System/Integer Model/Quadrotor Dynamic System/Rotational System/Equation3 ==
  x2 : Inport
  x4 : Inport  Port=2
  U4 : Inport  Port=3
  Gain : Gain  Commented=on  Gain=a3
  Gain1 : Gain  Commented=on  Gain=b3
  Gain2 : Gain
  Gain3 : Gain  Commented=on  Gain=c3
  Gain4 : Gain  Gain=Dis
  Integrator : Integrator
  Integrator1 : Integrator
  Math Function : Math  Operator=square  SignedPower=on
  Product{,1..3} (4 alike) : Product
  Sum : Sum  Inputs=|+++
  Sum1 : Sum
  x5 =Psi : Outport  VectorParamsAs1DForOutWhenUnconnected=off
  x6 : Outport  Port=2  VectorParamsAs1DForOutWhenUnconnected=off
  wires:
  Math Function/1 -> Product2/2  "x6^2"
  x2/1 -> Product/1
  Integrator/1 -> Math Function/1, x6/1, Integrator1/1
  U4/1 -> Product3/2
  Product3/1 -> Sum/3
  Product1/1 -> Sum/1  "a3 x2 x4"
  Product2/1 -> Sum/2  "b3 x6^2"
  Integrator1/1 -> x5 =Psi/1
  Product/1 -> Product1/2
  x4/1 -> Product/2
  Sum1/1 -> Integrator/1
  [Dphi3] -> Gain4/1
  Sum/1 -> Sum1/2
  Gain2/1 -> Sum1/1
  Gain4/1 -> Gain2/1
  [a3D] -> Product1/1
  [b3D] -> Product2/1
  [c3D] -> Product3/1

== system RobustFormationControl_IntegerModel_under_Dis/Integer Leader and four followers/Leader System/Integer Model/Quadrotor Dynamic System/Translational System/Equation4 ==
  U1 : Inport
  Ux : Inport  Port=2
  Divide : Product  Inputs=**  RndMeth=Zero  SaturateOnIntegerOverflow=on
  Divide1 : Product  Inputs=**  RndMeth=Zero  SaturateOnIntegerOverflow=on
  Gain : Gain  Commented=on  Gain=1/m
  Gain1 : Gain  Commented=on  Gain=a4
  Gain2 : Gain  Gain=1/m
  Gain3 : Gain  Gain=Dis
  Integrator : Integrator
  Integrator1 : Integrator
  Product : Product
  Sum : Sum  Inputs=|++
  Sum1 : Sum
  x7 = x : Outport  VectorParamsAs1DForOutWhenUnconnected=off
  x8 = xdot : Outport  Port=2  VectorParamsAs1DForOutWhenUnconnected=off
  wires:
  Integrator/1 -> Divide/1, x8 = xdot/1, Integrator1/1
  U1/1 -> Product/1
  Divide1/1 -> Sum/1  "U1 Ux / m"
  Divide/1 -> Sum/2  "a4 x8"
  Integrator1/1 -> x7 = x/1
  Product/1 -> Divide1/2
  Ux/1 -> Product/2
  Sum/1 -> Sum1/2
  Sum1/1 -> Integrator/1
  [Dpx] -> Gain3/1
  Gain2/1 -> Sum1/1
  [a4D] -> Divide/2
  [b4D] -> Divide1/1
  Gain3/1 -> Gain2/1

== system RobustFormationControl_IntegerModel_under_Dis/Integer Leader and four followers/Leader System/Integer Model/Quadrotor Dynamic System/Translational System/Equation5 ==
  U1 : Inport
  Uy : Inport  Port=2
  Divide : Product  Inputs=**  RndMeth=Zero  SaturateOnIntegerOverflow=on
  Divide1 : Product  Inputs=**  RndMeth=Zero  SaturateOnIntegerOverflow=on
  Gain : Gain  Commented=on  Gain=1/m
  Gain1 : Gain  Commented=on  Gain=a5
  Gain2 : Gain  Gain=1/m
  Gain3 : Gain  Commented=on  Gain=0
  Gain4 : Gain  Gain=Dis
  Integrator : Integrator
  Integrator1 : Integrator
  Product : Product
  Sum : Sum  Inputs=|++
  Sum1 : Sum
  x9 = y : Outport  VectorParamsAs1DForOutWhenUnconnected=off
  x10 = ydot : Outport  Port=2  VectorParamsAs1DForOutWhenUnconnected=off
  wires:
  Integrator/1 -> Divide/2, x10 = ydot/1, Integrator1/1
  U1/1 -> Product/1
  Divide1/1 -> Sum/1  "U1 Ux / m"
  Divide/1 -> Sum/2  "a4 x10"
  Integrator1/1 -> x9 = y/1
  Product/1 -> Divide1/2
  Uy/1 -> Product/2
  [a5D] -> Divide/1
  [b5D] -> Divide1/1
  Sum/1 -> Sum1/2
  Sum1/1 -> Integrator/1
  Gain2/1 -> Sum1/1
  [Dpy] -> Gain4/1
  Gain4/1 -> Gain2/1

== system RobustFormationControl_IntegerModel_under_Dis/Integer Leader and four followers/Leader System/Integer Model/Quadrotor Dynamic System/Translational System/Equation6 ==
  U1 : Inport
  x1 : Inport  Port=2
  x3 : Inport  Port=3
  Constant : Constant  Value=g
  Divide : Product  Inputs=**  RndMeth=Zero  SaturateOnIntegerOverflow=on
  Divide1 : Product  Inputs=**  RndMeth=Zero  SaturateOnIntegerOverflow=on
  Gain : Gain  Commented=on  Gain=1/m
  Gain1 : Gain  Commented=on  Gain=a6
  Gain2 : Gain  Gain=1/m
  Gain3 : Gain  Gain=Dis
  Integrator : Integrator
  Integrator1 : Integrator
  Product : Product
  Product1 : Product
  Sum : Sum  Inputs=|++-
  Sum1 : Sum
  Trigonometric Function : Trigonometry  Operator=cos
  Trigonometric Function1 : Trigonometry  Operator=cos
  x11 = z : Outport  VectorParamsAs1DForOutWhenUnconnected=off
  x12 = zdot : Outport  Port=2  VectorParamsAs1DForOutWhenUnconnected=off
  wires:
  U1/1 -> Product/1
  Divide1/1 -> Sum/1  "U1 cx1 cx3  / m"
  Divide/1 -> Sum/2  "a6 x12"
  Integrator1/1 -> x11 = z/1
  Product/1 -> Divide1/2
  Product1/1 -> Product/2
  Trigonometric Function/1 -> Product1/1
  Trigonometric Function1/1 -> Product1/2
  x1/1 -> Trigonometric Function/1
  x3/1 -> Trigonometric Function1/1
  Constant/1 -> Sum/3
  Integrator/1 -> Divide/2, x12 = zdot/1, Integrator1/1
  [a6D] -> Divide/1
  [b6D] -> Divide1/1
  Sum1/1 -> Integrator/1
  [Dpz] -> Gain3/1
  Sum/1 -> Sum1/2
  Gain2/1 -> Sum1/1
  Gain3/1 -> Gain2/1

== matlab function RobustFormationControl_IntegerModel_under_Dis/Integer Leader and four followers/Leader System/Stochastic Disturbances/Dphi2/MATLAB Function ==
  data: t input; Dphi2 output
function Dphi2 = fcn(t)

Dphi2 = 0.5*cos(0.5*t) + 1;

== matlab function RobustFormationControl_IntegerModel_under_Dis/Integer Leader and four followers/Leader System/Stochastic Disturbances/Dphi3/MATLAB Function ==
  data: t input; Dphi3 output
function Dphi3 = fcn(t)

Dphi3 = 0.05*cos(0.7*t) + 0.1;

== matlab function RobustFormationControl_IntegerModel_under_Dis/Integer Leader and four followers/Leader System/Stochastic Disturbances/Dpx/MATLAB Function ==
  data: t input; Dpx output
function Dpx = fcn(t)

Dpx = -0.08*sin(0.11*t - 3.0403) + 0.04*sin(0.5*t - 13.5) + 0.008*sin(1.6*t -15*pi) +0.006*sin(0.3*t - 8.6);

== matlab function RobustFormationControl_IntegerModel_under_Dis/Integer Leader and four followers/Leader System/Stochastic Disturbances/Dpy/MATLAB Function ==
  data: t input; Dpy output
function Dpy = fcn(t)

Dpy = 0.05*sin(0.4*t) + 0.05*cos(0.7*t);

== matlab function RobustFormationControl_IntegerModel_under_Dis/Integer Leader and four followers/Leader System/Stochastic Disturbances/Dpz/MATLAB Function ==
  data: t input; Dpz output
function Dpz = fcn(t)

Dpz = 0.05*sin(0.7*t) + 0.07*cos(0.3*t);

== matlab function RobustFormationControl_IntegerModel_under_Dis/Integer Leader and four followers/Leader System/Stochastic Disturbances/Dphi1/MATLAB Function ==
  data: t input; Dphi1 output
function Dphi1 = fcn(t)

Dphi1 = 0.5*cos(0.4*t) + 1;
